simulink model "Es2_simulink"  (R2025b)
settings: Solver=VariableStepAuto  StartTime=0.0  StopTime=10  RelTol=1e-3
settings Model: Creator=fsisa  LastModifiedBy=fsisa

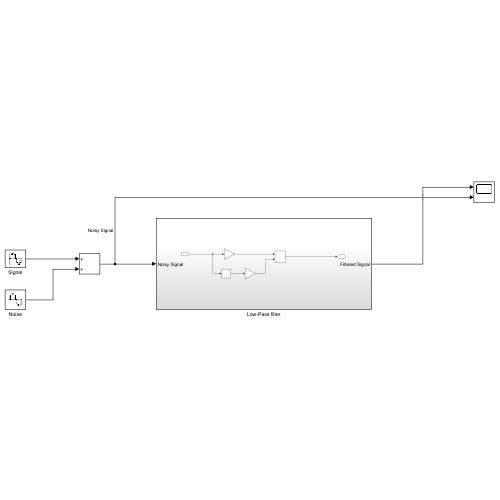
[thumbnail: Simulink's stored preview of the top-level diagram]
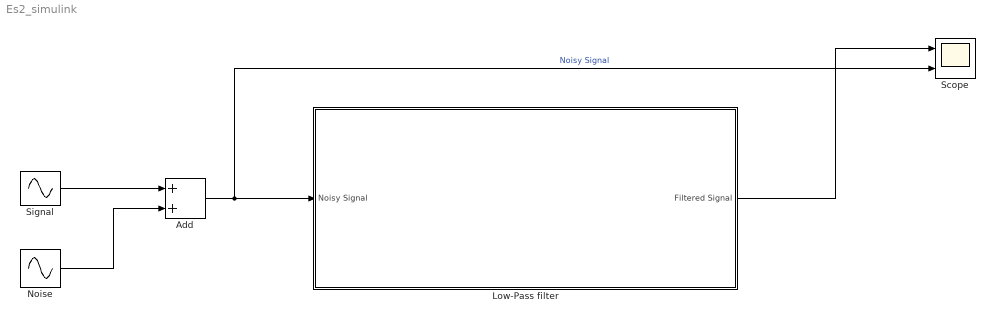
== system Es2_simulink ==
  Add : Sum
  Low-Pass filter : Subsystem
  Noise : Sin  Amplitude=2.5  Frequency=18  SampleTime=0.2
  Scope : Scope  NumInputPorts=2
      settings: ActiveDisplayYMinimum=-1  ActiveDisplayYMaximum=1
  Signal : Sin  Amplitude=10  SampleTime=0.2
  wires:
  Signal/1 -> Add/1
  Noise/1 -> Add/2
  Add/1 -> Scope/2, Low-Pass filter/1(Noisy Signal)  "Noisy Signal"
  Low-Pass filter/1(Filtered Signal) -> Scope/1

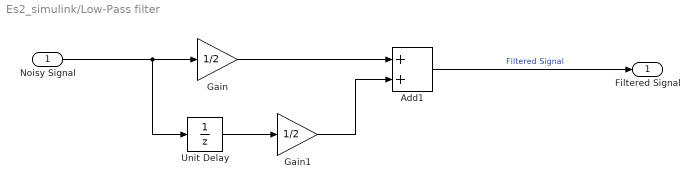
== system Es2_simulink/Low-Pass filter ==
  Noisy Signal : Inport
  Add1 : Sum
  Gain : Gain  Gain=1/2
  Gain1 : Gain  Gain=1/2
  Unit Delay : UnitDelay  SampleTime=-1  HasFrameUpgradeWarning=on
  Filtered Signal : Outport
  wires:
  Gain1/1 -> Add1/2
  Gain/1 -> Add1/1
  Unit Delay/1 -> Gain1/1
  Noisy Signal/1 -> Unit Delay/1, Gain/1
  Add1/1 -> Filtered Signal/1  "Filtered Signal"
